simulink model "DU_LUN_CHE_z_pid"  (R2023a)
settings: Solver=VariableStepAuto  StartTime=0.0  StopTime=10  RelTol=1e-3
undefined symbols (not defined in the file): X, Y, Z
libraries: sm_lib x77, nesl_utility x10, slpidlib x6, simulink x3
(part 2 of 3)

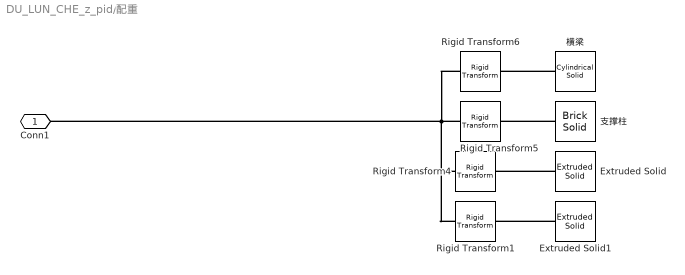
== system DU_LUN_CHE_z_pid/配重 ==
  Extruded Solid : sm_lib/Body Elements/Extruded Solid  GraphicAmbientColor=[0.15 0.15 0.15 1.0]  BasedOnType=Density  CenterOfMass=[0 0 0]  CenterOfMassUnits=m  GraphicDiffuseColor=[1.0 0.2 0.2]  ExportConvexHullGeometry=off  ExtrusionCrossSection=[0 10; -10 0; -3 0; -3 -15; 3 -15; 3 0; 10 0]  ExtrusionCrossSectionUnits=cm  Density=1000  DensityUnits=kg/m^3  DoExposeReferenceFrame=on  GraphicEmissiveColor=[0.0 0.0 0.0 1.0]  ExportEntireGeometry=off  ExtrusionLength=5  ExtrusionLengthUnits=cm  ExtrusionType=General  SerializedFrames=<Frames/>  MarkerShape=Sphere  MarkerSize=10  GraphicType=FromGeometry  InertiaType=PointMass  Mass=1  MassUnits=g  MomentsOfInertia=[1 1 1]  MomentsOfInertiaUnits=kg*m^2  PolygonNumSides=3  GraphicOpacity=0.9  PolygonOuterRadius=1  PolygonOuterRadiusUnits=m  ProductsOfInertia=[0 0 0]  ProductsOfInertiaUnits=kg*m^2  GraphicShininess=75  GraphicSpecularColor=[0.5 0.5 0.5 1.0]  GraphicVisPropType=SimpleVisualProperties
  Extruded Solid1 : sm_lib/Body Elements/Extruded Solid  GraphicAmbientColor=[0.15 0.15 0.15 1.0]  BasedOnType=Density  CenterOfMass=[0 0 0]  CenterOfMassUnits=m  GraphicDiffuseColor=[1.0 0.2 0.2]  ExportConvexHullGeometry=off  ExtrusionCrossSection=[0 10; -10 0; -3 0; -3 -15; 3 -15; 3 0; 10 0]  ExtrusionCrossSectionUnits=cm  Density=1000  DensityUnits=kg/m^3  DoExposeReferenceFrame=on  GraphicEmissiveColor=[0.0 0.0 0.0 1.0]  ExportEntireGeometry=off  ExtrusionLength=5  ExtrusionLengthUnits=cm  ExtrusionType=General  SerializedFrames=<Frames/>  MarkerShape=Sphere  MarkerSize=10  GraphicType=FromGeometry  InertiaType=PointMass  Mass=2  MassUnits=g  MomentsOfInertia=[1 1 1]  MomentsOfInertiaUnits=kg*m^2  PolygonNumSides=3  GraphicOpacity=0.9  PolygonOuterRadius=1  PolygonOuterRadiusUnits=m  ProductsOfInertia=[0 0 0]  ProductsOfInertiaUnits=kg*m^2  GraphicShininess=75  GraphicSpecularColor=[0.5 0.5 0.5 1.0]  GraphicVisPropType=SimpleVisualProperties
  Rigid Transform1 : sm_lib/Frames and Transforms/Rigid Transform  TranslationMethod=Cartesian  TranslationStandardOffset=0  TranslationStandardOffsetUnits=cm  TranslationStandardAxis=+Z  TranslationCartesianOffset=[55 10 00]  TranslationCartesianOffsetUnits=cm  TranslationROffset=0  TranslationROffsetUnits=m  TranslationZOffset=0  TranslationZOffsetUnits=m  TranslationThetaOffset=0  TranslationThetaOffsetUnits=deg  RotationMethod=RotationSequence  RotationAngleUnits=deg  RotationStandardAxis=+Z  RotationAngle=0.0  RotationArbitraryAxis=[0 0 1]  FollAlignAxisA=+X  BaseAlignAxisA=+Y  FollAlignAxisB=+Y  BaseAlignAxisB=+Z  RotationSequenceAxes=FollowerAxes  RotationSequence=XYZ  RotationSequenceAngles=[0 0 0]  RotationSequenceAnglesUnits=deg  RotationMatrix=[1 0 0; 0 1 0; 0 0 1]  Quaternion=[1 0 0 0]
  Rigid Transform4 : sm_lib/Frames and Transforms/Rigid Transform  TranslationMethod=Cartesian  TranslationStandardOffset=0  TranslationStandardOffsetUnits=cm  TranslationStandardAxis=+Z  TranslationCartesianOffset=[55 -20 00]  TranslationCartesianOffsetUnits=cm  TranslationROffset=0  TranslationROffsetUnits=m  TranslationZOffset=0  TranslationZOffsetUnits=m  TranslationThetaOffset=0  TranslationThetaOffsetUnits=deg  RotationMethod=RotationSequence  RotationAngleUnits=deg  RotationStandardAxis=+Z  RotationAngle=0.0  RotationArbitraryAxis=[0 0 1]  FollAlignAxisA=+X  BaseAlignAxisA=+Y  FollAlignAxisB=+Y  BaseAlignAxisB=+Z  RotationSequenceAxes=FollowerAxes  RotationSequence=XYZ  RotationSequenceAngles=[0 0 0]  RotationSequenceAnglesUnits=deg  RotationMatrix=[1 0 0; 0 1 0; 0 0 1]  Quaternion=[1 0 0 0]
  Rigid Transform5 : sm_lib/Frames and Transforms/Rigid Transform  TranslationMethod=Cartesian  TranslationStandardOffset=0  TranslationStandardOffsetUnits=cm  TranslationStandardAxis=+Z  TranslationCartesianOffset=[50 0 00]  TranslationCartesianOffsetUnits=cm  TranslationROffset=0  TranslationROffsetUnits=m  TranslationZOffset=0  TranslationZOffsetUnits=m  TranslationThetaOffset=0  TranslationThetaOffsetUnits=deg  RotationMethod=RotationSequence  RotationAngleUnits=deg  RotationStandardAxis=+Z  RotationAngle=0.0  RotationArbitraryAxis=[0 0 1]  FollAlignAxisA=+X  BaseAlignAxisA=+Y  FollAlignAxisB=+Y  BaseAlignAxisB=+Z  RotationSequenceAxes=FollowerAxes  RotationSequence=XYZ  RotationSequenceAngles=[0 0 0]  RotationSequenceAnglesUnits=deg  RotationMatrix=[1 0 0; 0 1 0; 0 0 1]  Quaternion=[1 0 0 0]
  Rigid Transform6 : sm_lib/Frames and Transforms/Rigid Transform  TranslationMethod=Cartesian  TranslationStandardOffset=0  TranslationStandardOffsetUnits=cm  TranslationStandardAxis=+Z  TranslationCartesianOffset=[70 0 00]  TranslationCartesianOffsetUnits=cm  TranslationROffset=0  TranslationROffsetUnits=m  TranslationZOffset=0  TranslationZOffsetUnits=m  TranslationThetaOffset=0  TranslationThetaOffsetUnits=deg  RotationMethod=RotationSequence  RotationAngleUnits=deg  RotationStandardAxis=+Z  RotationAngle=0.0  RotationArbitraryAxis=[0 0 1]  FollAlignAxisA=+X  BaseAlignAxisA=+Y  FollAlignAxisB=+Y  BaseAlignAxisB=+Z  RotationSequenceAxes=FollowerAxes  RotationSequence=XYZ  RotationSequenceAngles=[90 0 0]  RotationSequenceAnglesUnits=deg  RotationMatrix=[1 0 0; 0 1 0; 0 0 1]  Quaternion=[1 0 0 0]
  支撑柱 : sm_lib/Body Elements/Brick Solid  GraphicAmbientColor=[0.15 0.15 0.15 1.0]  BasedOnType=Mass  BrickDimensions=[50 10 10]  BrickDimensionsUnits=cm  CenterOfMass=[0 0 0]  CenterOfMassUnits=m  GraphicDiffuseColor=[0.0 0.4 0.4]  Density=1000  DensityUnits=kg/m^3  DoExposeReferenceFrame=on  GraphicEmissiveColor=[0.0 0.0 0.0 1.0]  ExportEntireGeometry=off  SerializedFrames=<Frames/>  MarkerShape=Sphere  MarkerSize=10  GraphicType=FromGeometry  InertiaType=CalculateFromGeometry  Mass=200  MassUnits=g  MomentsOfInertia=[1 1 1]  MomentsOfInertiaUnits=kg*m^2  GraphicOpacity=0.8  ProductsOfInertia=[0 0 0]  ProductsOfInertiaUnits=kg*m^2  GraphicShininess=75  GraphicSpecularColor=[0.5 0.5 0.5 1.0]  GraphicVisPropType=SimpleVisualProperties
  横梁 : sm_lib/Body Elements/Cylindrical Solid  GraphicAmbientColor=[0.15 0.15 0.15 1.0]  BasedOnType=Mass  CenterOfMass=[0 0 0]  CenterOfMassUnits=m  GraphicDiffuseColor=[0.2 0.2 1.0]  CylinderLength=100  CylinderLengthUnits=cm  CylinderRadius=7  CylinderRadiusUnits=cm  Density=1000  DensityUnits=kg/m^3  DoExposeReferenceFrame=on  GraphicEmissiveColor=[0.0 0.0 0.0 1.0]  ExportEntireGeometry=off  SerializedFrames=<Frames/>  MarkerShape=Sphere  MarkerSize=10  GraphicType=FromGeometry  InertiaType=CalculateFromGeometry  Mass=500  MassUnits=g  MomentsOfInertia=[1 1 1]  MomentsOfInertiaUnits=kg*m^2  GraphicOpacity=1  ProductsOfInertia=[0 0 0]  ProductsOfInertiaUnits=kg*m^2  GraphicShininess=75  GraphicSpecularColor=[0.5 0.5 0.5 1.0]  GraphicVisPropType=SimpleVisualProperties
  Conn1 : PMIOPort  Side=Left
  connections:
  Rigid Transform6/RConn1 -- Rigid Transform1/RConn1 -- Rigid Transform4/RConn1 -- Conn1/RConn1 -- Rigid Transform5/RConn1
  支撑柱/RConn1 -- Rigid Transform5/LConn1
  Extruded Solid/RConn1 -- Rigid Transform4/LConn1
  横梁/RConn1 -- Rigid Transform6/LConn1
  Extruded Solid1/RConn1 -- Rigid Transform1/LConn1

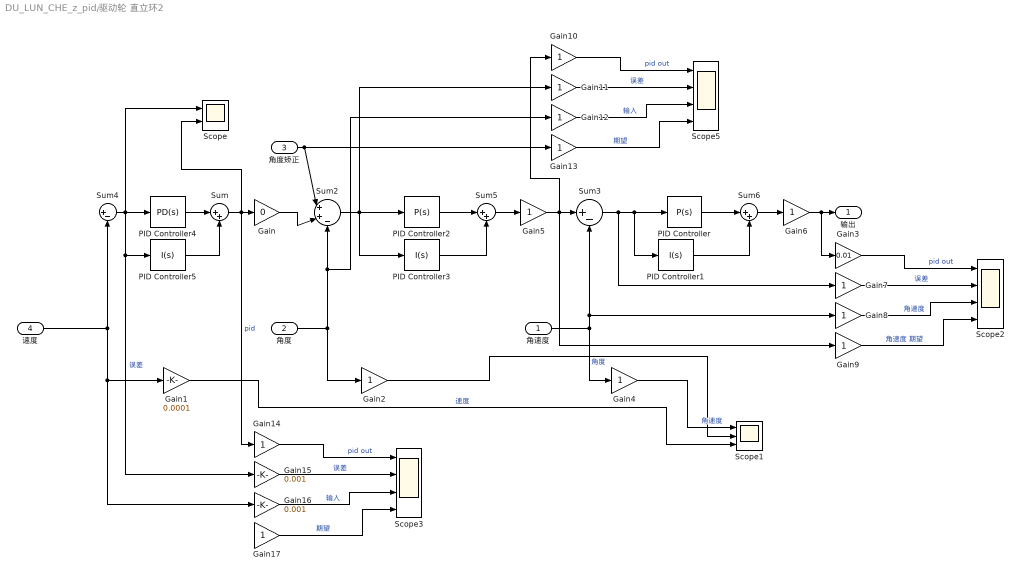
== system DU_LUN_CHE_z_pid/驱动轮 直立环2 ==
  角速度 : Inport
  角度 : Inport  Port=2
  角度矫正 : Inport  Port=3
  速度 : Inport  Port=4
  Gain : Gain  Gain=0
  Gain1 : Gain  Gain=0.0001
  Gain{2,4..14,17} (13 alike) : Gain
  Gain15 : Gain  Gain=0.001
  Gain16 : Gain  Gain=0.001
  Gain3 : Gain  Gain=0.01
  PID Controller : slpidlib/PID Controller  Controller=P  Form=Parallel  TimeDomain=Continuous-time  UseExternalTs=off  SampleTime=-1  IntegratorMethod=Forward Euler  FilterMethod=Forward Euler  ControllerParametersSource=internal  P=1  I=1  UseKiTs=off  D=0  N=100  UseFilter=on  TunerSelectOption=Transfer Function Based (PID Tuner App)  InitialConditionSource=internal  InitialConditionForIntegrator=0  InitialConditionForFilter=0  DifferentiatorICPrevScaledInput=0  ExternalReset=none  TrackingMode=off  Kt=1  LimitOutput=on  SatLimitsSource=internal  UpperSaturationLimit=800  LowerSaturationLimit=-800  LinearizeAsGain=on  AntiWindupMode=none  Kb=1  LimitIntegrator=off  UpperIntegratorSaturationLimit=inf  LowerIntegratorSaturationLimit=-inf  POutMin=[]  POutMax=[]  IOutMin=[]  IOutMax=[]  DOutMin=[]  DOutMax=[]  NOutMin=[]  NOutMax=[]  SumOutMin=[]  SumOutMax=[]  SaturationOutMin=[]  SaturationOutMax=[]  PParamMin=[]  PParamMax=[]  IParamMin=[]  IParamMax=[]  DParamMin=[]  DParamMax=[]  NParamMin=[]  NParamMax=[]  KbParamMin=[]  KbParamMax=[]  KtParamMin=[]  KtParamMax=[]  KbOutMin=[]  KbOutMax=[]  KtOutMin=[]  KtOutMax=[]  IntegratorOutMin=[]  IntegratorOutMax=[]  FilterOutMin=[]  FilterOutMax=[]  SumI1OutMin=[]  SumI1OutMax=[]  SumI2OutMin=[]  SumI2OutMax=[]  SumI3OutMin=[]  SumI3OutMax=[]  SumI4OutMin=[]  SumI4OutMax=[]  SumDOutMin=[]  SumDOutMax=[]  DifferentiatorOutMin=[]  DifferentiatorOutMax=[]  FilterDiffOutCoefMin=[]  FilterDiffOutCoefMax=[]  ReciprocalOutMin=[]  ReciprocalOutMax=[]  SumDenOutMin=[]  SumDenOutMax=[]  SumNumOutMin=[]  SumNumOutMax=[]  DivideOutMin=[]  DivideOutMax=[]  UdiffTsProdOutMin=[]  UdiffTsProdOutMax=[]  NTsProdOutMin=[]  NTsProdOutMax=[]  UintegralTsProdOutMin=[]  UintegralTsProdOutMax=[]  UngainTsProdOutMin=[]  UngainTsProdOutMax=[]  ClampingZeroOutDataTypeStr=Inherit: Inherit via back propagation  ClampingZeroOutMin=[]  ClampingZeroOutMax=[]  FilterDenConstantOutDataTypeStr=Inherit: Inherit via back propagation  FilterDenConstantOutMin=[]  FilterDenConstantOutMax=[]  PCopyOutDataTypeStr=Inherit: Inherit via back propagation  PCopyOutMin=[]  PCopyOutMax=[]  NCopyOutDataTypeStr=Inherit: Inherit via back propagation  NCopyOutMin=[]  NCopyOutMax=[]  IntegratorContinuousStateAttributes=''  IntegratorStateMustResolveToSignalObject=off  IntegratorRTWStateStorageClass=Auto  FilterContinuousStateAttributes=''  FilterStateMustResolveToSignalObject=off  FilterRTWStateStorageClass=Auto  ParallelPVariant=InternalParameters  IdealPVariant=Disabled  IVariant=Disabled  DVariant=Disabled  IntegratorVariant=Disabled  SatVariant=Enabled  AWVariant=Disabled  PCopyVariant=Disabled  TRVariant=Disabled  FdbkBlocksVariant=Forward  IdealPFdbkVariant=Disabled  SatFdbkVariant=Disabled  DerivativeFilterVariant=Disabled  NVariant=Disabled  NCopyVariant=Disabled_SignalSpec  FilterICVariant=Disabled  IntegratorICVariant=Disabled  ExternalResetVariant=Disabled  TRSumVariant=Passthrough  SumFdbkVariant=Disabled  SumVariant=Passthrough_P  TsampFilterVariant=InternalTs  TsampNgainVariant=Passthrough  TsampIntegralVariant=Disabled_SignalSpec  ExternalSaturationOutDataTypeStr=Inherit: Same as second input
  PID Controller1 : slpidlib/PID Controller  Controller=I  Form=Parallel  TimeDomain=Continuous-time  UseExternalTs=off  SampleTime=-1  IntegratorMethod=Forward Euler  FilterMethod=Forward Euler  ControllerParametersSource=internal  P=1  I=1  UseKiTs=off  D=0  N=100  UseFilter=on  TunerSelectOption=Transfer Function Based (PID Tuner App)  InitialConditionSource=internal  InitialConditionForIntegrator=0  InitialConditionForFilter=0  DifferentiatorICPrevScaledInput=0  ExternalReset=none  TrackingMode=off  Kt=1  LimitOutput=on  SatLimitsSource=internal  UpperSaturationLimit=1  LowerSaturationLimit=-1  LinearizeAsGain=on  AntiWindupMode=none  Kb=1  LimitIntegrator=off  UpperIntegratorSaturationLimit=inf  LowerIntegratorSaturationLimit=-inf  POutMin=[]  POutMax=[]  IOutMin=[]  IOutMax=[]  DOutMin=[]  DOutMax=[]  NOutMin=[]  NOutMax=[]  SumOutMin=[]  SumOutMax=[]  SaturationOutMin=[]  SaturationOutMax=[]  PParamMin=[]  PParamMax=[]  IParamMin=[]  IParamMax=[]  DParamMin=[]  DParamMax=[]  NParamMin=[]  NParamMax=[]  KbParamMin=[]  KbParamMax=[]  KtParamMin=[]  KtParamMax=[]  KbOutMin=[]  KbOutMax=[]  KtOutMin=[]  KtOutMax=[]  IntegratorOutMin=[]  IntegratorOutMax=[]  FilterOutMin=[]  FilterOutMax=[]  SumI1OutMin=[]  SumI1OutMax=[]  SumI2OutMin=[]  SumI2OutMax=[]  SumI3OutMin=[]  SumI3OutMax=[]  SumI4OutMin=[]  SumI4OutMax=[]  SumDOutMin=[]  SumDOutMax=[]  DifferentiatorOutMin=[]  DifferentiatorOutMax=[]  FilterDiffOutCoefMin=[]  FilterDiffOutCoefMax=[]  ReciprocalOutMin=[]  ReciprocalOutMax=[]  SumDenOutMin=[]  SumDenOutMax=[]  SumNumOutMin=[]  SumNumOutMax=[]  DivideOutMin=[]  DivideOutMax=[]  UdiffTsProdOutMin=[]  UdiffTsProdOutMax=[]  NTsProdOutMin=[]  NTsProdOutMax=[]  UintegralTsProdOutMin=[]  UintegralTsProdOutMax=[]  UngainTsProdOutMin=[]  UngainTsProdOutMax=[]  ClampingZeroOutDataTypeStr=Inherit: Inherit via back propagation  ClampingZeroOutMin=[]  ClampingZeroOutMax=[]  FilterDenConstantOutDataTypeStr=Inherit: Inherit via back propagation  FilterDenConstantOutMin=[]  FilterDenConstantOutMax=[]  PCopyOutDataTypeStr=Inherit: Inherit via back propagation  PCopyOutMin=[]  PCopyOutMax=[]  NCopyOutDataTypeStr=Inherit: Inherit via back propagation  NCopyOutMin=[]  NCopyOutMax=[]  IntegratorContinuousStateAttributes=''  IntegratorStateMustResolveToSignalObject=off  IntegratorRTWStateStorageClass=Auto  FilterContinuousStateAttributes=''  FilterStateMustResolveToSignalObject=off  FilterRTWStateStorageClass=Auto  ParallelPVariant=Disabled  IdealPVariant=Disabled  IVariant=InternalParameters  DVariant=Disabled  IntegratorVariant=Continuous  SatVariant=Enabled  AWVariant=Passthrough  PCopyVariant=Disabled  TRVariant=Disabled  FdbkBlocksVariant=Forward  IdealPFdbkVariant=Disabled  SatFdbkVariant=Disabled  DerivativeFilterVariant=Disabled  NVariant=Disabled  NCopyVariant=Disabled_SignalSpec  FilterICVariant=Disabled  IntegratorICVariant=InternalICs  ExternalResetVariant=Disabled  TRSumVariant=Passthrough  SumFdbkVariant=Disabled  SumVariant=Passthrough_I  TsampFilterVariant=InternalTs  TsampNgainVariant=Passthrough  TsampIntegralVariant=Disabled_SignalSpec  ExternalSaturationOutDataTypeStr=Inherit: Same as second input
  PID Controller2 : slpidlib/PID Controller  Controller=P  Form=Parallel  TimeDomain=Continuous-time  UseExternalTs=off  SampleTime=-1  IntegratorMethod=Forward Euler  FilterMethod=Forward Euler  ControllerParametersSource=internal  P=1  I=1  UseKiTs=off  D=0  N=100  UseFilter=on  TunerSelectOption=Transfer Function Based (PID Tuner App)  InitialConditionSource=internal  InitialConditionForIntegrator=0  InitialConditionForFilter=0  DifferentiatorICPrevScaledInput=0  ExternalReset=none  TrackingMode=off  Kt=1  LimitOutput=on  SatLimitsSource=internal  UpperSaturationLimit=5  LowerSaturationLimit=-5  LinearizeAsGain=on  AntiWindupMode=none  Kb=1  LimitIntegrator=off  UpperIntegratorSaturationLimit=inf  LowerIntegratorSaturationLimit=-inf  POutMin=[]  POutMax=[]  IOutMin=[]  IOutMax=[]  DOutMin=[]  DOutMax=[]  NOutMin=[]  NOutMax=[]  SumOutMin=[]  SumOutMax=[]  SaturationOutMin=[]  SaturationOutMax=[]  PParamMin=[]  PParamMax=[]  IParamMin=[]  IParamMax=[]  DParamMin=[]  DParamMax=[]  NParamMin=[]  NParamMax=[]  KbParamMin=[]  KbParamMax=[]  KtParamMin=[]  KtParamMax=[]  KbOutMin=[]  KbOutMax=[]  KtOutMin=[]  KtOutMax=[]  IntegratorOutMin=[]  IntegratorOutMax=[]  FilterOutMin=[]  FilterOutMax=[]  SumI1OutMin=[]  SumI1OutMax=[]  SumI2OutMin=[]  SumI2OutMax=[]  SumI3OutMin=[]  SumI3OutMax=[]  SumI4OutMin=[]  SumI4OutMax=[]  SumDOutMin=[]  SumDOutMax=[]  DifferentiatorOutMin=[]  DifferentiatorOutMax=[]  FilterDiffOutCoefMin=[]  FilterDiffOutCoefMax=[]  ReciprocalOutMin=[]  ReciprocalOutMax=[]  SumDenOutMin=[]  SumDenOutMax=[]  SumNumOutMin=[]  SumNumOutMax=[]  DivideOutMin=[]  DivideOutMax=[]  UdiffTsProdOutMin=[]  UdiffTsProdOutMax=[]  NTsProdOutMin=[]  NTsProdOutMax=[]  UintegralTsProdOutMin=[]  UintegralTsProdOutMax=[]  UngainTsProdOutMin=[]  UngainTsProdOutMax=[]  ClampingZeroOutDataTypeStr=Inherit: Inherit via back propagation  ClampingZeroOutMin=[]  ClampingZeroOutMax=[]  FilterDenConstantOutDataTypeStr=Inherit: Inherit via back propagation  FilterDenConstantOutMin=[]  FilterDenConstantOutMax=[]  PCopyOutDataTypeStr=Inherit: Inherit via back propagation  PCopyOutMin=[]  PCopyOutMax=[]  NCopyOutDataTypeStr=Inherit: Inherit via back propagation  NCopyOutMin=[]  NCopyOutMax=[]  IntegratorContinuousStateAttributes=''  IntegratorStateMustResolveToSignalObject=off  IntegratorRTWStateStorageClass=Auto  FilterContinuousStateAttributes=''  FilterStateMustResolveToSignalObject=off  FilterRTWStateStorageClass=Auto  ParallelPVariant=InternalParameters  IdealPVariant=Disabled  IVariant=Disabled  DVariant=Disabled  IntegratorVariant=Disabled  SatVariant=Enabled  AWVariant=Disabled  PCopyVariant=Disabled  TRVariant=Disabled  FdbkBlocksVariant=Forward  IdealPFdbkVariant=Disabled  SatFdbkVariant=Disabled  DerivativeFilterVariant=Disabled  NVariant=Disabled  NCopyVariant=Disabled_SignalSpec  FilterICVariant=Disabled  IntegratorICVariant=Disabled  ExternalResetVariant=Disabled  TRSumVariant=Passthrough  SumFdbkVariant=Disabled  SumVariant=Passthrough_P  TsampFilterVariant=InternalTs  TsampNgainVariant=Passthrough  TsampIntegralVariant=Disabled_SignalSpec  ExternalSaturationOutDataTypeStr=Inherit: Same as second input
  PID Controller3 : slpidlib/PID Controller  Controller=I  Form=Parallel  TimeDomain=Continuous-time  UseExternalTs=off  SampleTime=-1  IntegratorMethod=Forward Euler  FilterMethod=Forward Euler  ControllerParametersSource=internal  P=1  I=0  UseKiTs=off  D=0  N=100  UseFilter=on  TunerSelectOption=Transfer Function Based (PID Tuner App)  InitialConditionSource=internal  InitialConditionForIntegrator=0  InitialConditionForFilter=0  DifferentiatorICPrevScaledInput=0  ExternalReset=none  TrackingMode=off  Kt=1  LimitOutput=on  SatLimitsSource=internal  UpperSaturationLimit=100  LowerSaturationLimit=-100  LinearizeAsGain=on  AntiWindupMode=none  Kb=1  LimitIntegrator=off  UpperIntegratorSaturationLimit=inf  LowerIntegratorSaturationLimit=-inf  POutMin=[]  POutMax=[]  IOutMin=[]  IOutMax=[]  DOutMin=[]  DOutMax=[]  NOutMin=[]  NOutMax=[]  SumOutMin=[]  SumOutMax=[]  SaturationOutMin=[]  SaturationOutMax=[]  PParamMin=[]  PParamMax=[]  IParamMin=[]  IParamMax=[]  DParamMin=[]  DParamMax=[]  NParamMin=[]  NParamMax=[]  KbParamMin=[]  KbParamMax=[]  KtParamMin=[]  KtParamMax=[]  KbOutMin=[]  KbOutMax=[]  KtOutMin=[]  KtOutMax=[]  IntegratorOutMin=[]  IntegratorOutMax=[]  FilterOutMin=[]  FilterOutMax=[]  SumI1OutMin=[]  SumI1OutMax=[]  SumI2OutMin=[]  SumI2OutMax=[]  SumI3OutMin=[]  SumI3OutMax=[]  SumI4OutMin=[]  SumI4OutMax=[]  SumDOutMin=[]  SumDOutMax=[]  DifferentiatorOutMin=[]  DifferentiatorOutMax=[]  FilterDiffOutCoefMin=[]  FilterDiffOutCoefMax=[]  ReciprocalOutMin=[]  ReciprocalOutMax=[]  SumDenOutMin=[]  SumDenOutMax=[]  SumNumOutMin=[]  SumNumOutMax=[]  DivideOutMin=[]  DivideOutMax=[]  UdiffTsProdOutMin=[]  UdiffTsProdOutMax=[]  NTsProdOutMin=[]  NTsProdOutMax=[]  UintegralTsProdOutMin=[]  UintegralTsProdOutMax=[]  UngainTsProdOutMin=[]  UngainTsProdOutMax=[]  ClampingZeroOutDataTypeStr=Inherit: Inherit via back propagation  ClampingZeroOutMin=[]  ClampingZeroOutMax=[]  FilterDenConstantOutDataTypeStr=Inherit: Inherit via back propagation  FilterDenConstantOutMin=[]  FilterDenConstantOutMax=[]  PCopyOutDataTypeStr=Inherit: Inherit via back propagation  PCopyOutMin=[]  PCopyOutMax=[]  NCopyOutDataTypeStr=Inherit: Inherit via back propagation  NCopyOutMin=[]  NCopyOutMax=[]  IntegratorContinuousStateAttributes=''  IntegratorStateMustResolveToSignalObject=off  IntegratorRTWStateStorageClass=Auto  FilterContinuousStateAttributes=''  FilterStateMustResolveToSignalObject=off  FilterRTWStateStorageClass=Auto  ParallelPVariant=Disabled  IdealPVariant=Disabled  IVariant=InternalParameters  DVariant=Disabled  IntegratorVariant=Continuous  SatVariant=Enabled  AWVariant=Passthrough  PCopyVariant=Disabled  TRVariant=Disabled  FdbkBlocksVariant=Forward  IdealPFdbkVariant=Disabled  SatFdbkVariant=Disabled  DerivativeFilterVariant=Disabled  NVariant=Disabled  NCopyVariant=Disabled_SignalSpec  FilterICVariant=Disabled  IntegratorICVariant=InternalICs  ExternalResetVariant=Disabled  TRSumVariant=Passthrough  SumFdbkVariant=Disabled  SumVariant=Passthrough_I  TsampFilterVariant=InternalTs  TsampNgainVariant=Passthrough  TsampIntegralVariant=Disabled_SignalSpec  ExternalSaturationOutDataTypeStr=Inherit: Same as second input
  PID Controller4 : slpidlib/PID Controller  Controller=PD  Form=Parallel  TimeDomain=Continuous-time  UseExternalTs=off  SampleTime=-1  IntegratorMethod=Forward Euler  FilterMethod=Forward Euler  ControllerParametersSource=internal  P=0  I=1  UseKiTs=off  D=0  N=100  UseFilter=on  TunerSelectOption=Transfer Function Based (PID Tuner App)  InitialConditionSource=internal  InitialConditionForIntegrator=0  InitialConditionForFilter=0  DifferentiatorICPrevScaledInput=0  ExternalReset=none  TrackingMode=off  Kt=1  LimitOutput=on  SatLimitsSource=internal  UpperSaturationLimit=1  LowerSaturationLimit=-1  LinearizeAsGain=on  AntiWindupMode=none  Kb=1  LimitIntegrator=off  UpperIntegratorSaturationLimit=inf  LowerIntegratorSaturationLimit=-inf  POutMin=[]  POutMax=[]  IOutMin=[]  IOutMax=[]  DOutMin=[]  DOutMax=[]  NOutMin=[]  NOutMax=[]  SumOutMin=[]  SumOutMax=[]  SaturationOutMin=[]  SaturationOutMax=[]  PParamMin=[]  PParamMax=[]  IParamMin=[]  IParamMax=[]  DParamMin=[]  DParamMax=[]  NParamMin=[]  NParamMax=[]  KbParamMin=[]  KbParamMax=[]  KtParamMin=[]  KtParamMax=[]  KbOutMin=[]  KbOutMax=[]  KtOutMin=[]  KtOutMax=[]  IntegratorOutMin=[]  IntegratorOutMax=[]  FilterOutMin=[]  FilterOutMax=[]  SumI1OutMin=[]  SumI1OutMax=[]  SumI2OutMin=[]  SumI2OutMax=[]  SumI3OutMin=[]  SumI3OutMax=[]  SumI4OutMin=[]  SumI4OutMax=[]  SumDOutMin=[]  SumDOutMax=[]  DifferentiatorOutMin=[]  DifferentiatorOutMax=[]  FilterDiffOutCoefMin=[]  FilterDiffOutCoefMax=[]  ReciprocalOutMin=[]  ReciprocalOutMax=[]  SumDenOutMin=[]  SumDenOutMax=[]  SumNumOutMin=[]  SumNumOutMax=[]  DivideOutMin=[]  DivideOutMax=[]  UdiffTsProdOutMin=[]  UdiffTsProdOutMax=[]  NTsProdOutMin=[]  NTsProdOutMax=[]  UintegralTsProdOutMin=[]  UintegralTsProdOutMax=[]  UngainTsProdOutMin=[]  UngainTsProdOutMax=[]  ClampingZeroOutDataTypeStr=Inherit: Inherit via back propagation  ClampingZeroOutMin=[]  ClampingZeroOutMax=[]  FilterDenConstantOutDataTypeStr=Inherit: Inherit via back propagation  FilterDenConstantOutMin=[]  FilterDenConstantOutMax=[]  PCopyOutDataTypeStr=Inherit: Inherit via back propagation  PCopyOutMin=[]  PCopyOutMax=[]  NCopyOutDataTypeStr=Inherit: Inherit via back propagation  NCopyOutMin=[]  NCopyOutMax=[]  IntegratorContinuousStateAttributes=''  IntegratorStateMustResolveToSignalObject=off  IntegratorRTWStateStorageClass=Auto  FilterContinuousStateAttributes=''  FilterStateMustResolveToSignalObject=off  FilterRTWStateStorageClass=Auto  ParallelPVariant=InternalParameters  IdealPVariant=Disabled  IVariant=Disabled  DVariant=InternalParameters  IntegratorVariant=Disabled  SatVariant=Enabled  AWVariant=Disabled  PCopyVariant=Disabled  TRVariant=Disabled  FdbkBlocksVariant=Forward  IdealPFdbkVariant=Disabled  SatFdbkVariant=Disabled  DerivativeFilterVariant=ContFilter  NVariant=InternalParameters  NCopyVariant=Disabled  FilterICVariant=InternalICsFilter  IntegratorICVariant=Disabled  ExternalResetVariant=Disabled  TRSumVariant=Passthrough  SumFdbkVariant=Disabled  SumVariant=Sum_PD  TsampFilterVariant=InternalTs  TsampNgainVariant=Passthrough  TsampIntegralVariant=Disabled_SignalSpec  ExternalSaturationOutDataTypeStr=Inherit: Same as second input
  PID Controller5 : slpidlib/PID Controller  Controller=I  Form=Parallel  TimeDomain=Continuous-time  UseExternalTs=off  SampleTime=-1  IntegratorMethod=Forward Euler  FilterMethod=Forward Euler  ControllerParametersSource=internal  P=1  I=0  UseKiTs=off  D=0  N=100  UseFilter=on  TunerSelectOption=Transfer Function Based (PID Tuner App)  InitialConditionSource=internal  InitialConditionForIntegrator=0  InitialConditionForFilter=0  DifferentiatorICPrevScaledInput=0  ExternalReset=none  TrackingMode=off  Kt=1  LimitOutput=on  SatLimitsSource=internal  UpperSaturationLimit=1  LowerSaturationLimit=-1  LinearizeAsGain=on  AntiWindupMode=none  Kb=1  LimitIntegrator=off  UpperIntegratorSaturationLimit=inf  LowerIntegratorSaturationLimit=-inf  POutMin=[]  POutMax=[]  IOutMin=[]  IOutMax=[]  DOutMin=[]  DOutMax=[]  NOutMin=[]  NOutMax=[]  SumOutMin=[]  SumOutMax=[]  SaturationOutMin=[]  SaturationOutMax=[]  PParamMin=[]  PParamMax=[]  IParamMin=[]  IParamMax=[]  DParamMin=[]  DParamMax=[]  NParamMin=[]  NParamMax=[]  KbParamMin=[]  KbParamMax=[]  KtParamMin=[]  KtParamMax=[]  KbOutMin=[]  KbOutMax=[]  KtOutMin=[]  KtOutMax=[]  IntegratorOutMin=[]  IntegratorOutMax=[]  FilterOutMin=[]  FilterOutMax=[]  SumI1OutMin=[]  SumI1OutMax=[]  SumI2OutMin=[]  SumI2OutMax=[]  SumI3OutMin=[]  SumI3OutMax=[]  SumI4OutMin=[]  SumI4OutMax=[]  SumDOutMin=[]  SumDOutMax=[]  DifferentiatorOutMin=[]  DifferentiatorOutMax=[]  FilterDiffOutCoefMin=[]  FilterDiffOutCoefMax=[]  ReciprocalOutMin=[]  ReciprocalOutMax=[]  SumDenOutMin=[]  SumDenOutMax=[]  SumNumOutMin=[]  SumNumOutMax=[]  DivideOutMin=[]  DivideOutMax=[]  UdiffTsProdOutMin=[]  UdiffTsProdOutMax=[]  NTsProdOutMin=[]  NTsProdOutMax=[]  UintegralTsProdOutMin=[]  UintegralTsProdOutMax=[]  UngainTsProdOutMin=[]  UngainTsProdOutMax=[]  ClampingZeroOutDataTypeStr=Inherit: Inherit via back propagation  ClampingZeroOutMin=[]  ClampingZeroOutMax=[]  FilterDenConstantOutDataTypeStr=Inherit: Inherit via back propagation  FilterDenConstantOutMin=[]  FilterDenConstantOutMax=[]  PCopyOutDataTypeStr=Inherit: Inherit via back propagation  PCopyOutMin=[]  PCopyOutMax=[]  NCopyOutDataTypeStr=Inherit: Inherit via back propagation  NCopyOutMin=[]  NCopyOutMax=[]  IntegratorContinuousStateAttributes=''  IntegratorStateMustResolveToSignalObject=off  IntegratorRTWStateStorageClass=Auto  FilterContinuousStateAttributes=''  FilterStateMustResolveToSignalObject=off  FilterRTWStateStorageClass=Auto  ParallelPVariant=Disabled  IdealPVariant=Disabled  IVariant=InternalParameters  DVariant=Disabled  IntegratorVariant=Continuous  SatVariant=Enabled  AWVariant=Passthrough  PCopyVariant=Disabled  TRVariant=Disabled  FdbkBlocksVariant=Forward  IdealPFdbkVariant=Disabled  SatFdbkVariant=Disabled  DerivativeFilterVariant=Disabled  NVariant=Disabled  NCopyVariant=Disabled_SignalSpec  FilterICVariant=Disabled  IntegratorICVariant=InternalICs  ExternalResetVariant=Disabled  TRSumVariant=Passthrough  SumFdbkVariant=Disabled  SumVariant=Passthrough_I  TsampFilterVariant=InternalTs  TsampNgainVariant=Passthrough  TsampIntegralVariant=Disabled_SignalSpec  ExternalSaturationOutDataTypeStr=Inherit: Same as second input
  Scope : Scope  NumInputPorts=2
  Scope1 : Scope  NumInputPorts=3
  Scope2 : Scope  NumInputPorts=4
  Scope3 : Scope  NumInputPorts=4
  Scope5 : Scope  NumInputPorts=4
  Sum : Sum  Inputs=|++
  Sum2 : Sum  Inputs=|++-
  Sum3 : Sum  Inputs=|+-
  Sum4 : Sum  Inputs=|+-
  Sum5 : Sum  Inputs=|++
  Sum6 : Sum  Inputs=|++
  输出 : Outport
  wires:
  Gain16/1 -> Scope3/3  "输入"
  Gain15/1 -> Scope3/2  "误差"
  Gain17/1 -> Scope3/4  "期望"
  Gain14/1 -> Scope3/1  "pid out"
  Gain12/1 -> Scope5/3  "输入"
  角度/1 -> Sum2/3, Gain12/1, Gain2/1
  Gain/1 -> Sum2/2
  Gain5/1 -> Sum3/1, Gain10/1, Gain9/1
  Gain10/1 -> Scope5/1  "pid out"
  Gain13/1 -> Scope5/4  "期望"
  Sum2/1 -> PID Controller2/1, PID Controller3/1, Gain11/1
  Gain11/1 -> Scope5/2  "误差"
  Gain9/1 -> Scope2/4  "角速度 期望"
  Gain8/1 -> Scope2/3  "角速度"
  Gain7/1 -> Scope2/2  "误差"
  Sum3/1 -> PID Controller/1, PID Controller1/1, Gain7/1
  Gain3/1 -> Scope2/1  "pid out"
  Gain1/1 -> Scope1/3  "速度"
  Gain2/1 -> Scope1/2  "角度"
  Gain4/1 -> Scope1/1  "角速度"
  PID Controller4/1 -> Sum/1
  Sum4/1 -> PID Controller4/1, PID Controller5/1, Gain15/1, Scope/1  "误差"
  角度矫正/1 -> Sum2/1, Gain13/1
  速度/1 -> Sum4/2, Gain1/1, Gain16/1
  PID Controller3/1 -> Sum5/2
  PID Controller1/1 -> Sum6/2
  Sum/1 -> Scope/2, Gain/1, Gain14/1  "pid"
  PID Controller/1 -> Sum6/1
  Sum6/1 -> Gain6/1
  Gain6/1 -> 输出/1, Gain3/1
  PID Controller5/1 -> Sum/2
  角速度/1 -> Sum3/2, Gain8/1, Gain4/1
  Sum5/1 -> Gain5/1
  PID Controller2/1 -> Sum5/1

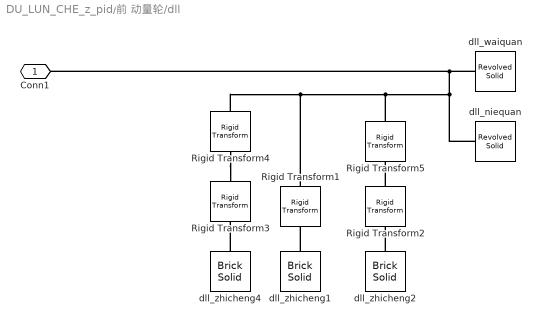
== system DU_LUN_CHE_z_pid/前 动量轮/dll ==
  Rigid Transform1 : sm_lib/Frames and Transforms/Rigid Transform  TranslationMethod=Cartesian  TranslationStandardOffset=0  TranslationStandardOffsetUnits=cm  TranslationStandardAxis=+Z  TranslationCartesianOffset=[17 0 -5]  TranslationCartesianOffsetUnits=cm  TranslationROffset=0  TranslationROffsetUnits=m  TranslationZOffset=0  TranslationZOffsetUnits=m  TranslationThetaOffset=0  TranslationThetaOffsetUnits=deg  RotationMethod=None  RotationAngleUnits=deg  RotationStandardAxis=+Z  RotationAngle=0.0  RotationArbitraryAxis=[0 0 1]  FollAlignAxisA=+X  BaseAlignAxisA=+Y  FollAlignAxisB=+Y  BaseAlignAxisB=+Z  RotationSequenceAxes=FollowerAxes  RotationSequence=XYX  RotationSequenceAngles=[0 0 0]  RotationSequenceAnglesUnits=deg  RotationMatrix=[1 0 0; 0 1 0; 0 0 1]  Quaternion=[1 0 0 0]
  Rigid Transform2 : sm_lib/Frames and Transforms/Rigid Transform  TranslationMethod=Cartesian  TranslationStandardOffset=0  TranslationStandardOffsetUnits=cm  TranslationStandardAxis=+Z  TranslationCartesianOffset=[17 0 -5]  TranslationCartesianOffsetUnits=cm  TranslationROffset=0  TranslationROffsetUnits=m  TranslationZOffset=0  TranslationZOffsetUnits=m  TranslationThetaOffset=0  TranslationThetaOffsetUnits=deg  RotationMethod=None  RotationAngleUnits=deg  RotationStandardAxis=+Z  RotationAngle=0.0  RotationArbitraryAxis=[0 0 1]  FollAlignAxisA=+X  BaseAlignAxisA=+Y  FollAlignAxisB=+Y  BaseAlignAxisB=+Z  RotationSequenceAxes=FollowerAxes  RotationSequence=XYX  RotationSequenceAngles=[0 0 0]  RotationSequenceAnglesUnits=deg  RotationMatrix=[1 0 0; 0 1 0; 0 0 1]  Quaternion=[1 0 0 0]
  Rigid Transform3 : sm_lib/Frames and Transforms/Rigid Transform  TranslationMethod=Cartesian  TranslationStandardOffset=0  TranslationStandardOffsetUnits=cm  TranslationStandardAxis=+Z  TranslationCartesianOffset=[17 0 -5]  TranslationCartesianOffsetUnits=cm  TranslationROffset=0  TranslationROffsetUnits=m  TranslationZOffset=0  TranslationZOffsetUnits=m  TranslationThetaOffset=0  TranslationThetaOffsetUnits=deg  RotationMethod=None  RotationAngleUnits=deg  RotationStandardAxis=+Z  RotationAngle=0.0  RotationArbitraryAxis=[0 0 1]  FollAlignAxisA=+X  BaseAlignAxisA=+Y  FollAlignAxisB=+Y  BaseAlignAxisB=+Z  RotationSequenceAxes=FollowerAxes  RotationSequence=XYX  RotationSequenceAngles=[0 0 0]  RotationSequenceAnglesUnits=deg  RotationMatrix=[1 0 0; 0 1 0; 0 0 1]  Quaternion=[1 0 0 0]
  Rigid Transform4 : sm_lib/Frames and Transforms/Rigid Transform  TranslationMethod=None  TranslationStandardOffset=0  TranslationStandardOffsetUnits=m  TranslationStandardAxis=+Z  TranslationCartesianOffset=[0 0 0]  TranslationCartesianOffsetUnits=m  TranslationROffset=0  TranslationROffsetUnits=m  TranslationZOffset=0  TranslationZOffsetUnits=m  TranslationThetaOffset=120  TranslationThetaOffsetUnits=rad  RotationMethod=RotationSequence  RotationAngleUnits=deg  RotationStandardAxis=+Z  RotationAngle=0.0  RotationArbitraryAxis=[0 0 1]  FollAlignAxisA=+X  BaseAlignAxisA=+Y  FollAlignAxisB=+Y  BaseAlignAxisB=+Z  RotationSequenceAxes=FollowerAxes  RotationSequence=YZY  RotationSequenceAngles=[0 180 0]  RotationSequenceAnglesUnits=rad  RotationMatrix=[1 0 0; 0 1 0; 0 0 1]  Quaternion=[1 0 0 0]
  Rigid Transform5 : sm_lib/Frames and Transforms/Rigid Transform  TranslationMethod=None  TranslationStandardOffset=0  TranslationStandardOffsetUnits=m  TranslationStandardAxis=+Z  TranslationCartesianOffset=[0 0 0]  TranslationCartesianOffsetUnits=m  TranslationROffset=0  TranslationROffsetUnits=m  TranslationZOffset=0  TranslationZOffsetUnits=m  TranslationThetaOffset=120  TranslationThetaOffsetUnits=rad  RotationMethod=RotationSequence  RotationAngleUnits=deg  RotationStandardAxis=+Z  RotationAngle=0.0  RotationArbitraryAxis=[0 0 1]  FollAlignAxisA=+X  BaseAlignAxisA=+Y  FollAlignAxisB=+Y  BaseAlignAxisB=+Z  RotationSequenceAxes=FollowerAxes  RotationSequence=YZY  RotationSequenceAngles=[0 -180 0]  RotationSequenceAnglesUnits=rad  RotationMatrix=[1 0 0; 0 1 0; 0 0 1]  Quaternion=[1 0 0 0]
  dll_niequan : sm_lib/Body Elements/Revolved Solid  GraphicAmbientColor=[0.15 0.15 0.15 1.0]  BasedOnType=Mass  CenterOfMass=[0 0 0]  CenterOfMassUnits=m  GraphicDiffuseColor=[0.8 0.2 0.0]  ExportConvexHullGeometry=off  Density=1000  DensityUnits=kg/m^3  DoExposeReferenceFrame=on  GraphicEmissiveColor=[0.0 0.0 0.0 1.0]  ExportEntireGeometry=off  SerializedFrames=<Frames/>  MarkerShape=Sphere  MarkerSize=10  GraphicType=FromGeometry  InertiaType=CalculateFromGeometry  Mass=0.1  MassUnits=kg  MomentsOfInertia=[1 1 1]  MomentsOfInertiaUnits=kg*m^2  GraphicOpacity=0.9  ProductsOfInertia=[0 0 0]  ProductsOfInertiaUnits=kg*m^2  RevolutionCrossSection=[5 10; 5 -0; 10 -0; 10 10]  RevolutionCrossSectionUnits=cm  RevolutionAngle=180  RevolutionAngleUnits=deg  RevolutionExtent=Full  GraphicShininess=75  GraphicSpecularColor=[0.5 0.5 0.5 1.0]  GraphicVisPropType=SimpleVisualProperties
  dll_waiquan : sm_lib/Body Elements/Revolved Solid  GraphicAmbientColor=[0.15 0.15 0.15 1.0]  BasedOnType=Mass  CenterOfMass=[0 0 0]  CenterOfMassUnits=m  GraphicDiffuseColor=[0.8 0.2 0.0]  ExportConvexHullGeometry=off  Density=1000  DensityUnits=kg/m^3  DoExposeReferenceFrame=on  GraphicEmissiveColor=[0.0 0.0 0.0 1.0]  ExportEntireGeometry=off  SerializedFrames=<Frames/>  MarkerShape=Sphere  MarkerSize=10  GraphicType=FromGeometry  InertiaType=CalculateFromGeometry  Mass=0.4  MassUnits=kg  MomentsOfInertia=[1 1 1]  MomentsOfInertiaUnits=kg*m^2  GraphicOpacity=0.9  ProductsOfInertia=[0 0 0]  ProductsOfInertiaUnits=kg*m^2  RevolutionCrossSection=[25 10; 25 -0; 35 -0; 35 10]  RevolutionCrossSectionUnits=cm  RevolutionAngle=180  RevolutionAngleUnits=deg  RevolutionExtent=Full  GraphicShininess=75  GraphicSpecularColor=[0.5 0.5 0.5 1.0]  GraphicVisPropType=SimpleVisualProperties
  dll_zhicheng1 : sm_lib/Body Elements/Brick Solid  GraphicAmbientColor=[0.15 0.15 0.15 1.0]  BasedOnType=Mass  BrickDimensions=[20 10 8]  BrickDimensionsUnits=cm  CenterOfMass=[0 0 0]  CenterOfMassUnits=m  GraphicDiffuseColor=[1.0 0.8 0.2]  Density=1000  DensityUnits=kg/m^3  DoExposeReferenceFrame=on  GraphicEmissiveColor=[0.0 0.0 0.0 1.0]  ExportEntireGeometry=off  SerializedFrames=<Frames/>  MarkerShape=Sphere  MarkerSize=10  GraphicType=FromGeometry  InertiaType=CalculateFromGeometry  Mass=0  MassUnits=g  MomentsOfInertia=[1 1 1]  MomentsOfInertiaUnits=kg*m^2  GraphicOpacity=0.7  ProductsOfInertia=[0 0 0]  ProductsOfInertiaUnits=kg*m^2  GraphicShininess=75  GraphicSpecularColor=[0.5 0.5 0.5 1.0]  GraphicVisPropType=SimpleVisualProperties
  dll_zhicheng2 : sm_lib/Body Elements/Brick Solid  GraphicAmbientColor=[0.15 0.15 0.15 1.0]  BasedOnType=Mass  BrickDimensions=[20 10 8]  BrickDimensionsUnits=cm  CenterOfMass=[0 0 0]  CenterOfMassUnits=m  GraphicDiffuseColor=[1.0 0.8 0.2]  Density=1000  DensityUnits=kg/m^3  DoExposeReferenceFrame=on  GraphicEmissiveColor=[0.0 0.0 0.0 1.0]  ExportEntireGeometry=off  SerializedFrames=<Frames/>  MarkerShape=Sphere  MarkerSize=10  GraphicType=FromGeometry  InertiaType=CalculateFromGeometry  Mass=0  MassUnits=g  MomentsOfInertia=[1 1 1]  MomentsOfInertiaUnits=kg*m^2  GraphicOpacity=0.7  ProductsOfInertia=[0 0 0]  ProductsOfInertiaUnits=kg*m^2  GraphicShininess=75  GraphicSpecularColor=[0.5 0.5 0.5 1.0]  GraphicVisPropType=SimpleVisualProperties
  dll_zhicheng4 : sm_lib/Body Elements/Brick Solid  GraphicAmbientColor=[0.15 0.15 0.15 1.0]  BasedOnType=Mass  BrickDimensions=[20 10 8]  BrickDimensionsUnits=cm  CenterOfMass=[0 0 0]  CenterOfMassUnits=m  GraphicDiffuseColor=[1.0 0.8 0.2]  Density=1000  DensityUnits=kg/m^3  DoExposeReferenceFrame=on  GraphicEmissiveColor=[0.0 0.0 0.0 1.0]  ExportEntireGeometry=off  SerializedFrames=<Frames/>  MarkerShape=Sphere  MarkerSize=10  GraphicType=FromGeometry  InertiaType=CalculateFromGeometry  Mass=0  MassUnits=g  MomentsOfInertia=[1 1 1]  MomentsOfInertiaUnits=kg*m^2  GraphicOpacity=0.7  ProductsOfInertia=[0 0 0]  ProductsOfInertiaUnits=kg*m^2  GraphicShininess=75  GraphicSpecularColor=[0.5 0.5 0.5 1.0]  GraphicVisPropType=SimpleVisualProperties
  Conn1 : PMIOPort  Side=Left
  connections:
  dll_zhicheng4/RConn1 -- Rigid Transform3/LConn1
  Rigid Transform4/RConn1 -- Rigid Transform1/RConn1 -- Rigid Transform5/RConn1 -- Conn1/RConn1 -- dll_waiquan/RConn1 -- dll_niequan/RConn1
  Rigid Transform2/RConn1 -- Rigid Transform5/LConn1
  Rigid Transform4/LConn1 -- Rigid Transform3/RConn1
  dll_zhicheng1/RConn1 -- Rigid Transform1/LConn1
  dll_zhicheng2/RConn1 -- Rigid Transform2/LConn1

== system DU_LUN_CHE_z_pid/前 动量轮/gan ==
  Brick Solid1 : sm_lib/Body Elements/Brick Solid  GraphicAmbientColor=[0.15 0.15 0.15 1.0]  BasedOnType=Mass  BrickDimensions=[60 10 10]  BrickDimensionsUnits=cm  CenterOfMass=[0 0 0]  CenterOfMassUnits=m  GraphicDiffuseColor=[1.0 0.0 1.0]  Density=1000  DensityUnits=kg/m^3  DoExposeReferenceFrame=on  GraphicEmissiveColor=[0.0 0.0 0.0 1.0]  ExportEntireGeometry=off  SerializedFrames=<Frames/>  MarkerShape=Sphere  MarkerSize=10  GraphicType=FromGeometry  InertiaType=CalculateFromGeometry  Mass=500  MassUnits=g  MomentsOfInertia=[1 1 1]  MomentsOfInertiaUnits=kg*m^2  GraphicOpacity=0.8  ProductsOfInertia=[0 0 0]  ProductsOfInertiaUnits=kg*m^2  GraphicShininess=75  GraphicSpecularColor=[0.5 0.5 0.5 1.0]  GraphicVisPropType=SimpleVisualProperties
  Revolved Solid : sm_lib/Body Elements/Revolved Solid  Commented=on  GraphicAmbientColor=[0.15 0.15 0.15 1.0]  BasedOnType=Mass  CenterOfMass=[0 0 0]  CenterOfMassUnits=m  GraphicDiffuseColor=[1.0 0.6 0.0]  ExportConvexHullGeometry=off  Density=1000  DensityUnits=kg/m^3  DoExposeReferenceFrame=on  GraphicEmissiveColor=[0.0 0.0 0.0 1.0]  ExportEntireGeometry=off  SerializedFrames=<Frames/>  MarkerShape=Sphere  MarkerSize=10  GraphicType=FromGeometry  InertiaType=CalculateFromGeometry  Mass=10  MassUnits=g  MomentsOfInertia=[1 1 1]  MomentsOfInertiaUnits=kg*m^2  GraphicOpacity=0.7  ProductsOfInertia=[0 0 0]  ProductsOfInertiaUnits=kg*m^2  RevolutionCrossSection=[10 10; 10 0; 15 10; 15 0]  RevolutionCrossSectionUnits=cm  RevolutionAngle=180  RevolutionAngleUnits=deg  RevolutionExtent=Full  GraphicShininess=75  GraphicSpecularColor=[0.5 0.5 0.5 1.0]  GraphicVisPropType=SimpleVisualProperties
  Rigid Transform1 : sm_lib/Frames and Transforms/Rigid Transform  TranslationMethod=Cartesian  TranslationStandardOffset=0  TranslationStandardOffsetUnits=cm  TranslationStandardAxis=+Z  TranslationCartesianOffset=[20 0 0]  TranslationCartesianOffsetUnits=cm  TranslationROffset=0  TranslationROffsetUnits=m  TranslationZOffset=0  TranslationZOffsetUnits=m  TranslationThetaOffset=0  TranslationThetaOffsetUnits=deg  RotationMethod=None  RotationAngleUnits=deg  RotationStandardAxis=+Z  RotationAngle=0.0  RotationArbitraryAxis=[0 0 1]  FollAlignAxisA=+X  BaseAlignAxisA=+Y  FollAlignAxisB=+Y  BaseAlignAxisB=+Z  RotationSequenceAxes=FollowerAxes  RotationSequence=XYX  RotationSequenceAngles=[0 0 0]  RotationSequenceAnglesUnits=deg  RotationMatrix=[1 0 0; 0 1 0; 0 0 1]  Quaternion=[1 0 0 0]
  Rigid Transform2 : sm_lib/Frames and Transforms/Rigid Transform  TranslationMethod=Cartesian  TranslationStandardOffset=0  TranslationStandardOffsetUnits=cm  TranslationStandardAxis=+Z  TranslationCartesianOffset=[40 0 5]  TranslationCartesianOffsetUnits=cm  TranslationROffset=0  TranslationROffsetUnits=m  TranslationZOffset=0  TranslationZOffsetUnits=m  TranslationThetaOffset=0  TranslationThetaOffsetUnits=deg  RotationMethod=None  RotationAngleUnits=deg  RotationStandardAxis=+Z  RotationAngle=0.0  RotationArbitraryAxis=[0 0 1]  FollAlignAxisA=+X  BaseAlignAxisA=+Y  FollAlignAxisB=+Y  BaseAlignAxisB=+Z  RotationSequenceAxes=FollowerAxes  RotationSequence=XYX  RotationSequenceAngles=[0 0 0]  RotationSequenceAnglesUnits=deg  RotationMatrix=[1 0 0; 0 1 0; 0 0 1]  Quaternion=[1 0 0 0]
  Rigid Transform3 : sm_lib/Frames and Transforms/Rigid Transform  TranslationMethod=Cartesian  TranslationStandardOffset=0  TranslationStandardOffsetUnits=cm  TranslationStandardAxis=+Z  TranslationCartesianOffset=[0 0 5]  TranslationCartesianOffsetUnits=cm  TranslationROffset=0  TranslationROffsetUnits=m  TranslationZOffset=0  TranslationZOffsetUnits=m  TranslationThetaOffset=0  TranslationThetaOffsetUnits=deg  RotationMethod=None  RotationAngleUnits=deg  RotationStandardAxis=+Z  RotationAngle=0.0  RotationArbitraryAxis=[0 0 1]  FollAlignAxisA=+X  BaseAlignAxisA=+Y  FollAlignAxisB=+Y  BaseAlignAxisB=+Z  RotationSequenceAxes=FollowerAxes  RotationSequence=XYX  RotationSequenceAngles=[0 0 0]  RotationSequenceAnglesUnits=deg  RotationMatrix=[1 0 0; 0 1 0; 0 0 1]  Quaternion=[1 0 0 0]
  Rigid Transform4 : sm_lib/Frames and Transforms/Rigid Transform  Commented=on  TranslationMethod=Cartesian  TranslationStandardOffset=0  TranslationStandardOffsetUnits=cm  TranslationStandardAxis=+Z  TranslationCartesianOffset=[00 0 0]  TranslationCartesianOffsetUnits=cm  TranslationROffset=0  TranslationROffsetUnits=m  TranslationZOffset=0  TranslationZOffsetUnits=m  TranslationThetaOffset=0  TranslationThetaOffsetUnits=deg  RotationMethod=None  RotationAngleUnits=deg  RotationStandardAxis=+Z  RotationAngle=0.0  RotationArbitraryAxis=[0 0 1]  FollAlignAxisA=+X  BaseAlignAxisA=+Y  FollAlignAxisB=+Y  BaseAlignAxisB=+Z  RotationSequenceAxes=FollowerAxes  RotationSequence=XYX  RotationSequenceAngles=[0 0 0]  RotationSequenceAnglesUnits=deg  RotationMatrix=[1 0 0; 0 1 0; 0 0 1]  Quaternion=[1 0 0 0]
  lianjeigan1 : sm_lib/Body Elements/Cylindrical Solid  GraphicAmbientColor=[0.15 0.15 0.15 1.0]  BasedOnType=Mass  CenterOfMass=[0 0 0]  CenterOfMassUnits=m  GraphicDiffuseColor=[0.0 0.6 1.0]  CylinderLength=13  CylinderLengthUnits=cm  CylinderRadius=13  CylinderRadiusUnits=cm  Density=1000  DensityUnits=g/cm^3  DoExposeReferenceFrame=on  GraphicEmissiveColor=[0.0 0.0 0.0 1.0]  ExportEntireGeometry=off  SerializedFrames=<Frames/>  MarkerShape=Sphere  MarkerSize=10  GraphicType=FromGeometry  InertiaType=CalculateFromGeometry  Mass=10  MassUnits=g  MomentsOfInertia=[1 1 1]  MomentsOfInertiaUnits=kg*m^2  GraphicOpacity=1  ProductsOfInertia=[0 0 0]  ProductsOfInertiaUnits=kg*m^2  GraphicShininess=75  GraphicSpecularColor=[0.5 0.5 0.5 1.0]  GraphicVisPropType=SimpleVisualProperties
  lianjeigan2 : sm_lib/Body Elements/Cylindrical Solid  GraphicAmbientColor=[0.15 0.15 0.15 1.0]  BasedOnType=Mass  CenterOfMass=[0 0 0]  CenterOfMassUnits=m  GraphicDiffuseColor=[0.0 0.6 0.4]  CylinderLength=18  CylinderLengthUnits=cm  CylinderRadius=6  CylinderRadiusUnits=cm  Density=1000  DensityUnits=g/cm^3  DoExposeReferenceFrame=on  GraphicEmissiveColor=[0.0 0.0 0.0 1.0]  ExportEntireGeometry=off  SerializedFrames=<Frames/>  MarkerShape=Sphere  MarkerSize=10  GraphicType=FromGeometry  InertiaType=CalculateFromGeometry  Mass=10  MassUnits=g  MomentsOfInertia=[1 1 1]  MomentsOfInertiaUnits=kg*m^2  GraphicOpacity=0.8  ProductsOfInertia=[0 0 0]  ProductsOfInertiaUnits=kg*m^2  GraphicShininess=75  GraphicSpecularColor=[0.5 0.5 0.5 1.0]  GraphicVisPropType=SimpleVisualProperties
  Conn1 : PMIOPort  Side=Left
  connections:
  lianjeigan1/RConn1 -- Rigid Transform1/RConn1 -- Rigid Transform3/LConn1
  Rigid Transform4/RConn1 -- Revolved Solid/RConn1
  Brick Solid1/RConn1 -- Rigid Transform1/LConn1 -- Rigid Transform2/RConn1
  Rigid Transform3/RConn1 -- lianjeigan2/RConn1
  Rigid Transform4/LConn1 -- Conn1/RConn1 -- Rigid Transform2/LConn1
